simulink model "buck 16v"  (R2021b)
settings: Solver=FixedStepDiscrete  StartTime=0.0  StopTime=0.2  FixedStep=2e-8  RelTol=1e-3
libraries: spsSeriesRLCBranchLib x3, simulink x2, spsCurrentMeasurementLib x1, spsDCVoltageSourceLib x1, spsDiodeLib x1, spsGroundLib x1, spsIdealSwitchLib x1, spsVoltageMeasurementLib x1, spspowerguiLib x1
settings Model: Creator=wu330  LastModifiedBy=wu330

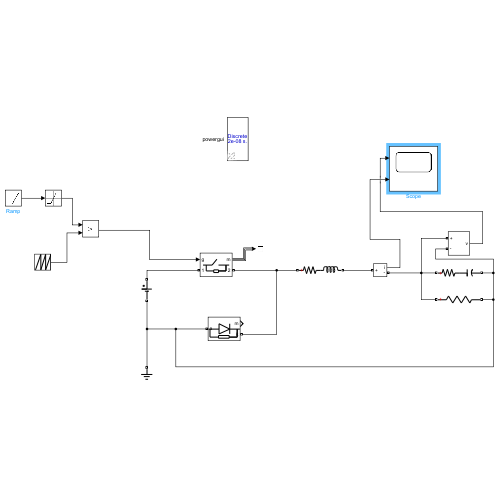
[thumbnail: Simulink's stored preview of the top-level diagram]
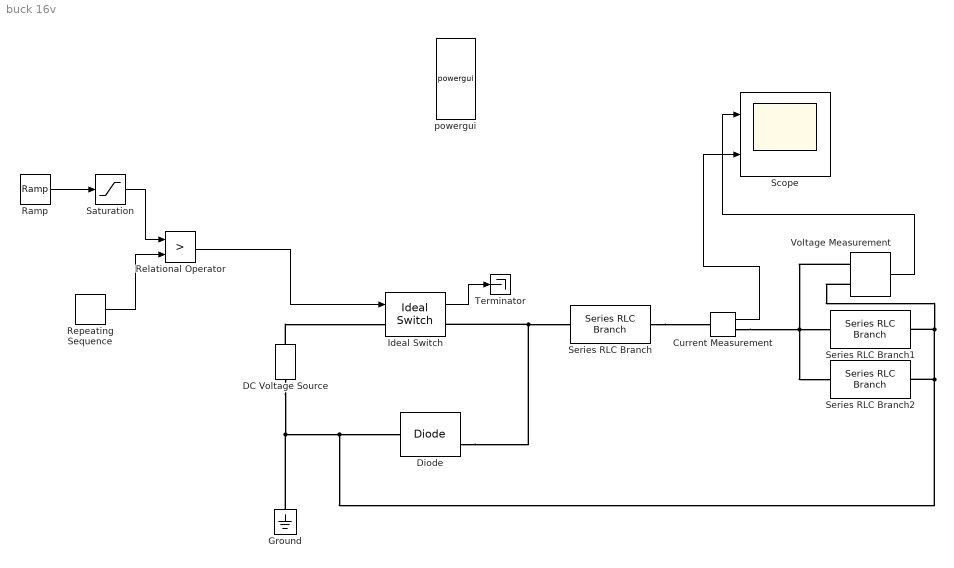
== system buck 16v ==
  Current Measurement : spsCurrentMeasurementLib/Current Measurement  PhasorSimulation=off  OutputType=Complex  PSBequivalent=0
  DC Voltage Source : spsDCVoltageSourceLib/DC Voltage Source  Amplitude=24  Measurements=None
  Diode : spsDiodeLib/Diode  Ron=0.001  Lon=0  Vf=0.5  IC=0  UseSnubber=0  Rs=500  Cs=250e-9  Measurements=on
  Ground : spsGroundLib/Ground  LConnTagsString=a
  Ideal Switch : spsIdealSwitchLib/Ideal Switch  Ron=0.01  Lon=0  IC=0  Rs=1e5  Cs=inf  Measurements=on
  Ramp : simulink/Sources/Ramp  slope=134  start=0  InitialOutput=0
  Relational Operator : RelationalOperator  Operator=>  OutDataTypeStr=boolean  RndMeth=Simplest
  Repeating Sequence : simulink/Sources/Repeating Sequence  rep_seq_t=[0 2e-6]  rep_seq_y=[0 1]
  Saturation : Saturate  UpperLimit=0.67  LowerLimit=0
  Scope : Scope  NumInputPorts=2
  Series RLC Branch : spsSeriesRLCBranchLib/Series RLC Branch  LConnTagsString=__new0  RConnTagsString=__new0  BranchType=RL  Resistance=0.074  Inductance=22e-6  SetiL0=on  InitialCurrent=0  Capacitance=1e-6  Setx0=off  InitialVoltage=0  Measurements=None
  Series RLC Branch1 : spsSeriesRLCBranchLib/Series RLC Branch  LConnTagsString=__new0  RConnTagsString=__new0  BranchType=RC  Resistance=0.03  Inductance=1e-3  SetiL0=off  InitialCurrent=0  Capacitance=220e-6  Setx0=on  InitialVoltage=0  Measurements=None
  Series RLC Branch2 : spsSeriesRLCBranchLib/Series RLC Branch  LConnTagsString=__new0  RConnTagsString=__new0  BranchType=R  Resistance=8  Inductance=1e-3  SetiL0=off  InitialCurrent=0  Capacitance=1e-6  Setx0=off  InitialVoltage=0  Measurements=None
  Terminator : Terminator
  Voltage Measurement : spsVoltageMeasurementLib/Voltage Measurement  PhasorSimulation=off  OutputType=Complex  PSBequivalent=0
  powergui : spspowerguiLib/powergui  Priority=1  SimulationMode=Discrete  SampleTime=2e-8  frequency=60  Iterations=50  frequencyindice=0  Pbase=100e6  ErrMax=1e-4  UnitsV=kV  UnitsW=MW  buscounter=0  FunctionMessages=off  echomessages=off  EnableUseOfTLC=off  CurrentSourceSwitches=off  DisableSnubberDevices=off  DisableRonSwitches=off  DisableVfSwitches=off  DisplayEquations=off  AutomaticDiscreteSolvers=off  SolverType=Tustin/Backward Euler (TBE)  Interpol=off  ExternalGateDelay=off  methode=off  Ts=100  x0status=blocks  SPID=on  SwTol=0  HookPort=off  NonlinearTolerance=1e-4  nMaxIteration=100  ContinueOnMaxIteration=off  RestoreLinks=warning  ResistiveCurrentMeasurement=off  Frange=[0:2:500]  Ylog=off  Xlog=on  ShowGrid=off  save=off  variable=ZData  structure=0  ZoomFFT=off  StartTime=0.0  cycles=1  DisplayStyle=1  fundamental=60  FreqAxis=off  MaxFrequency=1000  frequencyindicesteady=1  RmsSteady=1  display=off
  wires:
  Ideal Switch/1 -> Terminator/1
  Voltage Measurement/1 -> Scope/1
  Current Measurement/1 -> Scope/2
  Ramp/1 -> Saturation/1
  Saturation/1 -> Relational Operator/1
  Repeating Sequence/1 -> Relational Operator/2
  Relational Operator/1 -> Ideal Switch/1
  connections:
  DC Voltage Source/RConn1 -- Ideal Switch/LConn1
  Series RLC Branch/RConn1 -- Current Measurement/LConn1
  Current Measurement/RConn1 -- Series RLC Branch2/LConn1 -- Voltage Measurement/LConn1 -- Series RLC Branch1/LConn1
  DC Voltage Source/LConn1 -- Ground/LConn1 -- Voltage Measurement/LConn2 -- Series RLC Branch1/RConn1 -- Series RLC Branch2/RConn1 -- Diode/LConn1
  Diode/RConn1 -- Series RLC Branch/LConn1 -- Ideal Switch/RConn1
